simulink model "StarshipSystemModel"  (R2025b)
settings: Solver=VariableStepAuto  StartTime=0.0  StopTime=10.0  RelTol=1e-3
model workspace (MAT data in the model file):
  ActiveGNCMode : Simulink.Bus (value not decoded)
  AerodynamicControlCommand : Simulink.Bus (value not decoded)
  AerodynamicLoad : Simulink.Bus (value not decoded)
  AggregatedStream : Simulink.Bus (value not decoded)
  AllocatedEffectorDemand : Simulink.Bus (value not decoded)
  AttitudeControlDemand : Simulink.Bus (value not decoded)
  AttitudeGuidanceCommand : Simulink.Bus (value not decoded)
  AttitudeRateState : Simulink.Bus (value not decoded)
  AutogenousPressurantGas : Simulink.ConnectionBus (value not decoded)
  CandidateFaultIndication : Simulink.Bus (value not decoded)
  CombustionGasFeed : Simulink.ConnectionBus (value not decoded)
  CommandPathHealth : Simulink.Bus (value not decoded)
  ControlMode : Simulink.ValueType (value not decoded)
  DownlinkSignal : Simulink.Bus (value not decoded)
  ElectricalPower : Simulink.ConnectionBus (value not decoded)
  EngineTelemetry : Simulink.Bus (value not decoded)
  ExecutionContext : Simulink.Bus (value not decoded)
  FaultDiagnosisResult : Simulink.Bus (value not decoded)
  GNCDataContext : Simulink.Bus (value not decoded)
  GNCHealthState : Simulink.Bus (value not decoded)
  GNCStateEstimate : Simulink.Bus (value not decoded)
  GimbalAngle : Simulink.ValueType (value not decoded)
  GimbalMotion : Simulink.ConnectionBus (value not decoded)
  GroundCheckoutLink : Simulink.Bus (value not decoded)
  GroundPressurantSupply : Simulink.ConnectionBus (value not decoded)
  GuidanceConstraints : Simulink.Bus (value not decoded)
  GuidanceMode : Simulink.ValueType (value not decoded)
  LinkHealth : Simulink.Bus (value not decoded)
  LiquidPropellantFeed : Simulink.ConnectionBus (value not decoded)
  MechanicalMotion : Simulink.ConnectionBus (value not decoded)
  MechanismPosition : Simulink.Bus (value not decoded)
  ModeTransitionContext : Simulink.Bus (value not decoded)
  NavigationAidingData : Simulink.Bus (value not decoded)
  NavigationEstimate : Simulink.Bus (value not decoded)
  NavigationHealthStatus : Simulink.Bus (value not decoded)
  NavigationMeasurementSet : Simulink.Bus (value not decoded)
  PercentThrottle : Simulink.ValueType (value not decoded)
  PneumaticActuationGas : Simulink.ConnectionBus (value not decoded)
  PowerConversionStatus : Simulink.Bus (value not decoded)
  PowerDistributionStatus : Simulink.Bus (value not decoded)
  PowerHealthStatus : Simulink.Bus (value not decoded)
  PowerManagementCommand : Simulink.Bus (value not decoded)
  PowerStorageStatus : Simulink.Bus (value not decoded)
  ProtectedThermalState : Simulink.Bus (value not decoded)
  ProtectionIsolationStatus : Simulink.Bus (value not decoded)
  PurgeGasSupply : Simulink.ConnectionBus (value not decoded)
  RCSPulseCommand : Simulink.Bus (value not decoded)
  RCSTelemetry : Simulink.Bus (value not decoded)
  RFFeed : Simulink.ConnectionBus (value not decoded)
  RecoveryMechanismCommand : Simulink.Bus (value not decoded)
  RollThrottleBias : Simulink.ValueType (value not decoded)
  SafetyOverride : Simulink.ValueType (value not decoded)
  SafetyStateStatus : Simulink.Bus (value not decoded)
  ShapedControlDemand : Simulink.Bus (value not decoded)
  SpinStartIgniterGas : Simulink.ConnectionBus (value not decoded)
  StageMechanicalBoundary : Simulink.ConnectionBus (value not decoded)
  StructuralLoad : Simulink.ConnectionBus (value not decoded)
  StructureHealthStatus : Simulink.Bus (value not decoded)
  SubsystemHealthEvidence : Simulink.Bus (value not decoded)
  SubsystemStatusTelemetry : Simulink.Bus (value not decoded)
  TankTelemetry : Simulink.Bus (value not decoded)
  ThermalMonitoringCommand : Simulink.Bus (value not decoded)
  ThermalNetwork : Simulink.ConnectionBus (value not decoded)
  ThrustLoad : Simulink.ConnectionBus (value not decoded)
  TrajectoryGuidanceCommand : Simulink.Bus (value not decoded)
  TrajectoryReference : Simulink.Bus (value not decoded)
  TranslationalControlDemand : Simulink.Bus (value not decoded)
  TranslationalState : Simulink.Bus (value not decoded)
  UplinkSignal : Simulink.Bus (value not decoded)
  ValidatedControlDemand : Simulink.Bus (value not decoded)
  ValveCommand : Simulink.ValueType (value not decoded)
  VehicleStructureState : Simulink.Bus (value not decoded)
  VerifiedCommand : Simulink.Bus (value not decoded)
  VideoStream : Simulink.Bus (value not decoded)
undefined symbols (not defined in the file): ACR, ACT, ASM, ATM, BCR, BDQ, BDR, BDX, BEC, BFC, BHV, BIP, BLM, BNZ, BPI, BPR, BPV, BRX, BSM, BTA, BTP, BVC, BVE, BVV, CAA, CAM, CAS, CAT, CLM, COM, CRS, CTL, CTR, DAQ, ESC, EXT, FCR, FDB, FDE, FEX, FHI, FHM, FIC, FIS, FMG, FSC, GAP, GCM, GMD, GNC, GND, GPH, GTR, HDN, HIA, HSI, IF, INT, LOC, NAI ... (+45)
(part 6 of 8)

== system StarshipSystemModel/Starship/Thermal Protection/Thermal Barriers & Discontinuity Protection ==
  Bus Element In8 : Inport  PortName=IF-BTP-LOC-TBI-STP-01
  Bus Element In7 : Inport  Port=2  PortName=IF-BTP-FHI-TBI-INT-01
  Bus Element In6 : Inport  Port=3  PortName=IF-BTP-ACR-TBI-GAP-01
  Bus Element In5 : Inport  Port=4  PortName=IF-STP-LOC-TBI-STP-01
  Bus Element In4 : Inport  Port=5  PortName=IF-STP-CTL-TBI-CTL-01
  Bus Element In3 : Inport  Port=6  PortName=IF-STP-ACR-TBI-GAP-01
  Control-surface boundary / closeout protection : Subsystem
      settings: PortSchema="{\"entries\":[{\"content\":{\"headerSize\":26,\"margin\":15,\"minimumSpacing\":25,\"sides\":[{\"content\":{\"connectorIds\":[\"In1\"]},\"type\":\"ConnectorPlacement.EquallySpacedRectSide\",\"uuid\":\"e0cfb70a-2480-46ad-8838-78efdb61b60e\"},{\"content\":{\"connectorIds\":[\"Out1\"],\"side\":\"RIGHT\"},\"type\":\"ConnectorPlacement.EquallySpacedRectSide\",\"uuid\":\"0844e172-3ed8-42bd-94dc-a51d08e37039\"},{\"content\":{\"side\":\"TOP\"},\"type\":\"ConnectorPlacement.EquallySpacedRectSide\",\"uuid\":\"2415ea6e-ae7d-422f-a1cc-5a10cd0c87f7\"}]},\"type\":\"ConnectorPlacement.EquallySpacedConnector\",\"uuid\":\"814347a2-9201-4b2d-b96f-a93fca4a3c45\"}],\"packageUris\":[\"http://schema.mathworks.com/mf0/Connector/R2020b\"],\"version\":\"1.0\"}"
  Penetration and interface barriers : Subsystem
      settings: PortSchema="{\"entries\":[{\"content\":{\"headerSize\":26,\"margin\":15,\"minimumSpacing\":25,\"sides\":[{\"content\":{\"connectorIds\":[\"In1\"]},\"type\":\"ConnectorPlacement.EquallySpacedRectSide\",\"uuid\":\"e0cfb70a-2480-46ad-8838-78efdb61b60e\"},{\"content\":{\"connectorIds\":[\"Out1\"],\"side\":\"RIGHT\"},\"type\":\"ConnectorPlacement.EquallySpacedRectSide\",\"uuid\":\"0844e172-3ed8-42bd-94dc-a51d08e37039\"},{\"content\":{\"side\":\"TOP\"},\"type\":\"ConnectorPlacement.EquallySpacedRectSide\",\"uuid\":\"2415ea6e-ae7d-422f-a1cc-5a10cd0c87f7\"}]},\"type\":\"ConnectorPlacement.EquallySpacedConnector\",\"uuid\":\"814347a2-9201-4b2d-b96f-a93fca4a3c45\"}],\"packageUris\":[\"http://schema.mathworks.com/mf0/Connector/R2020b\"],\"version\":\"1.0\"}"
  Step / protrusion thermal management : Subsystem
      settings: PortSchema="{\"entries\":[{\"content\":{\"headerSize\":26,\"margin\":15,\"minimumSpacing\":25,\"sides\":[{\"content\":{\"connectorIds\":[\"In1\",\"In2\"]},\"type\":\"ConnectorPlacement.EquallySpacedRectSide\",\"uuid\":\"e0cfb70a-2480-46ad-8838-78efdb61b60e\"},{\"content\":{\"connectorIds\":[\"RConn1\"],\"side\":\"RIGHT\"},\"type\":\"ConnectorPlacement.EquallySpacedRectSide\",\"uuid\":\"0844e172-3ed8-42bd-94dc-a51d08e37039\"},{\"content\":{\"side\":\"TOP\"},\"type\":\"ConnectorPlacement.EquallySpacedRectSide\",\"uuid\":\"2415ea6e-ae7d-422f-a1cc-5a10cd0c87f7\"}]},\"type\":\"ConnectorPlacement.EquallySpacedConnector\",\"uuid\":\"814347a2-9201-4b2d-b96f-a93fca4a3c45\"}],\"packageUris\":[\"http://schema.mathworks.com/mf0/Connector/R2020b\"],\"version\":\"1.0\"}"
  Tile-gap / seam thermal protection : Subsystem
      settings: PortSchema="{\"entries\":[{\"content\":{\"headerSize\":26,\"margin\":15,\"minimumSpacing\":25,\"sides\":[{\"content\":{\"connectorIds\":[\"In1\",\"In2\"]},\"type\":\"ConnectorPlacement.EquallySpacedRectSide\",\"uuid\":\"e0cfb70a-2480-46ad-8838-78efdb61b60e\"},{\"content\":{\"connectorIds\":[\"Out1\"],\"side\":\"RIGHT\"},\"type\":\"ConnectorPlacement.EquallySpacedRectSide\",\"uuid\":\"0844e172-3ed8-42bd-94dc-a51d08e37039\"},{\"content\":{\"side\":\"TOP\"},\"type\":\"ConnectorPlacement.EquallySpacedRectSide\",\"uuid\":\"2415ea6e-ae7d-422f-a1cc-5a10cd0c87f7\"}]},\"type\":\"ConnectorPlacement.EquallySpacedConnector\",\"uuid\":\"814347a2-9201-4b2d-b96f-a93fca4a3c45\"}],\"packageUris\":[\"http://schema.mathworks.com/mf0/Connector/R2020b\"],\"version\":\"1.0\"}"
  IF-TBI-PRS-01 : PMIOPort  Side=Right  ConnectionType=Bus: ThermalNetwork
  Bus Element Out2 : Outport  PortName=IF-TBI-GAP-TMS-SNS-01
  Bus Element Out3 : Outport  Port=2  PortName=IF-TBI-INT-TMS-SNS-01
  Bus Element Out4 : Outport  Port=3  PortName=IF-TBI-CTL-TMS-SNS-01
  wires:
  Bus Element In4/1 -> Control-surface boundary / closeout protection/1(IF-STP-CTL-TBI-CTL-01)
  Bus Element In6/1 -> Tile-gap / seam thermal protection/1(IF-BTP-ACR-TBI-GAP-01)
  Bus Element In8/1 -> Step / protrusion thermal management/1(IF-BTP-LOC-TBI-STP-01)
  Bus Element In7/1 -> Penetration and interface barriers/1(IF-BTP-FHI-TBI-INT-01)
  Bus Element In3/1 -> Tile-gap / seam thermal protection/2(IF-STP-ACR-TBI-GAP-01)
  Bus Element In5/1 -> Step / protrusion thermal management/2(IF-STP-LOC-TBI-STP-01)
  Tile-gap / seam thermal protection/1(IF-TBI-GAP-TMS-SNS-01) -> Bus Element Out2/1
  Control-surface boundary / closeout protection/1(IF-TBI-CTL-TMS-SNS-01) -> Bus Element Out4/1
  Penetration and interface barriers/1(IF-TBI-INT-TMS-SNS-01) -> Bus Element Out3/1
  connections:
  IF-TBI-PRS-01/RConn1 -- Step / protrusion thermal management/RConn1

== system StarshipSystemModel/Starship/Thermal Protection/Thermal Monitoring & Assessment ==
  Bus Element In3 : Inport  PortName=IF-TBI-GAP-TMS-SNS-01
  Bus Element In4 : Inport  Port=2  PortName=IF-TBI-INT-TMS-SNS-01
  Bus Element In5 : Inport  Port=3  PortName=IF-TBI-CTL-TMS-SNS-01
  Bus Element In1 : Inport  Port=4  PortName=IF-GNC-TMS-01
  External thermal-observation data interface : Subsystem
      settings: PortSchema="{\"entries\":[{\"content\":{\"headerSize\":26,\"margin\":15,\"minimumSpacing\":25,\"sides\":[{\"content\":{},\"type\":\"ConnectorPlacement.EquallySpacedRectSide\",\"uuid\":\"e0cfb70a-2480-46ad-8838-78efdb61b60e\"},{\"content\":{\"connectorIds\":[\"Out1\"],\"side\":\"RIGHT\"},\"type\":\"ConnectorPlacement.EquallySpacedRectSide\",\"uuid\":\"0844e172-3ed8-42bd-94dc-a51d08e37039\"},{\"content\":{\"side\":\"TOP\"},\"type\":\"ConnectorPlacement.EquallySpacedRectSide\",\"uuid\":\"2415ea6e-ae7d-422f-a1cc-5a10cd0c87f7\"}]},\"type\":\"ConnectorPlacement.EquallySpacedConnector\",\"uuid\":\"814347a2-9201-4b2d-b96f-a93fca4a3c45\"}],\"packageUris\":[\"http://schema.mathworks.com/mf0/Connector/R2020b\"],\"version\":\"1.0\"}"
  TPS thermal sensors : Subsystem
      settings: PortSchema="{\"entries\":[{\"content\":{\"headerSize\":26,\"margin\":15,\"minimumSpacing\":25,\"sides\":[{\"content\":{\"connectorIds\":[\"In1\",\"In2\",\"In3\",\"In4\",\"LConn1\"]},\"type\":\"ConnectorPlacement.EquallySpacedRectSide\",\"uuid\":\"e0cfb70a-2480-46ad-8838-78efdb61b60e\"},{\"content\":{\"connectorIds\":[\"Out1\"],\"side\":\"RIGHT\"},\"type\":\"ConnectorPlacement.EquallySpacedRectSide\",\"uuid\":\"0844e172-3ed8-42bd-94dc-a51d08e37039\"},{\"content\":{\"side\":\"TOP\"},\"type\":\"ConnectorPlacement.EquallySpacedRectSide\",\"uuid\":\"2415ea6e-ae7d-422f-a1cc-5a10cd0c87f7\"}]},\"type\":\"ConnectorPlacement.EquallySpacedConnector\",\"uuid\":\"814347a2-9201-4b2d-b96f-a93fca4a3c45\"}],\"packageUris\":[\"http://schema.mathworks.com/mf0/Connector/R2020b\"],\"version\":\"1.0\"}"
  Thermal assessment / reconstruction function : Subsystem
      settings: PortSchema="{\"entries\":[{\"content\":{\"headerSize\":26,\"margin\":15,\"minimumSpacing\":25,\"sides\":[{\"content\":{\"connectorIds\":[\"In1\",\"In2\"]},\"type\":\"ConnectorPlacement.EquallySpacedRectSide\",\"uuid\":\"e0cfb70a-2480-46ad-8838-78efdb61b60e\"},{\"content\":{\"connectorIds\":[\"Out1\"],\"side\":\"RIGHT\"},\"type\":\"ConnectorPlacement.EquallySpacedRectSide\",\"uuid\":\"0844e172-3ed8-42bd-94dc-a51d08e37039\"},{\"content\":{\"side\":\"TOP\"},\"type\":\"ConnectorPlacement.EquallySpacedRectSide\",\"uuid\":\"2415ea6e-ae7d-422f-a1cc-5a10cd0c87f7\"}]},\"type\":\"ConnectorPlacement.EquallySpacedConnector\",\"uuid\":\"814347a2-9201-4b2d-b96f-a93fca4a3c45\"}],\"packageUris\":[\"http://schema.mathworks.com/mf0/Connector/R2020b\"],\"version\":\"1.0\"}"
  Thermal-data acquisition / telemetry path : Subsystem
      settings: PortSchema="{\"entries\":[{\"content\":{\"headerSize\":26,\"margin\":15,\"minimumSpacing\":25,\"sides\":[{\"content\":{\"connectorIds\":[\"In1\",\"In2\"]},\"type\":\"ConnectorPlacement.EquallySpacedRectSide\",\"uuid\":\"e0cfb70a-2480-46ad-8838-78efdb61b60e\"},{\"content\":{\"connectorIds\":[\"Out1\"],\"side\":\"RIGHT\"},\"type\":\"ConnectorPlacement.EquallySpacedRectSide\",\"uuid\":\"0844e172-3ed8-42bd-94dc-a51d08e37039\"},{\"content\":{\"side\":\"TOP\"},\"type\":\"ConnectorPlacement.EquallySpacedRectSide\",\"uuid\":\"2415ea6e-ae7d-422f-a1cc-5a10cd0c87f7\"}]},\"type\":\"ConnectorPlacement.EquallySpacedConnector\",\"uuid\":\"814347a2-9201-4b2d-b96f-a93fca4a3c45\"}],\"packageUris\":[\"http://schema.mathworks.com/mf0/Connector/R2020b\"],\"version\":\"1.0\"}"
  IF-PWR-TMS-01 : PMIOPort  Side=Left  ConnectionType=Bus: ElectricalPower
  Bus Element Out1 : Outport  PortName=IF-TMS-GNC-01
  Bus Element Out2 : Outport  Port=2  PortName=IF-TMS-BTA-01
  Bus Element Out3 : Outport  Port=3  PortName=IF-TMS-STA-01
  Bus Element Out4 : Outport  Port=4  PortName=IF-TMS-SAF-01
  wires:
  Bus Element In3/1 -> TPS thermal sensors/1(IF-TBI-GAP-TMS-SNS-01)
  Bus Element In4/1 -> TPS thermal sensors/2(IF-TBI-INT-TMS-SNS-01)
  Bus Element In5/1 -> TPS thermal sensors/3(IF-TBI-CTL-TMS-SNS-01)
  TPS thermal sensors/1(IF-TMS-SNS-DAQ-01) -> Thermal-data acquisition / telemetry path/1(IF-TMS-SNS-DAQ-01)
  Thermal-data acquisition / telemetry path/1(IF-TMS-DAQ-ASM-01) -> Thermal assessment / reconstruction function/1(IF-TMS-DAQ-ASM-01)
  Thermal assessment / reconstruction function/1(IF-TMS-ASM-DAQ-01) -> Thermal-data acquisition / telemetry path/2(IF-TMS-ASM-DAQ-01)
  External thermal-observation data interface/1(IF-TMS-EXT-ASM-01) -> Thermal assessment / reconstruction function/2(IF-TMS-EXT-ASM-01)
  Bus Element In1/1 -> TPS thermal sensors/4(IF-GNC-TMS-01)
  connections:
  IF-PWR-TMS-01/RConn1 -- TPS thermal sensors/LConn1

== system StarshipSystemModel/Starship/Communications/Booster/Command & Data Handling (C&DH) ==
  Bus Element In6 : Inport  PortName=IF-INT-BTA-01
  Bus Element In5 : Inport  Port=2  PortName=IF-TMS-BTA-01
  Bus Element In9 : Inport  Port=3  PortName=IF-BDQ-BCR-01
  Bus Element In8 : Inport  Port=4  PortName=IF-BDX-BLM-01
  Bus Element In7 : Inport  Port=5  PortName=IF-BRX-BLM-01
  Bus Element In3 : Inport  Port=6  PortName=IF-GNC-BTA-01
  Bus Element In2 : Inport  Port=7  PortName=IF-BPR-BTA-01
  Bus Element In1 : Inport  Port=8  PortName=IF-BEC-BTA-01
  Bus Element In4 : Inport  Port=9  PortName=IF-SAF-BTA-01
  Command decoder & router : Subsystem
      settings: PortSchema="{\"entries\":[{\"content\":{\"headerSize\":26,\"margin\":15,\"minimumSpacing\":25,\"sides\":[{\"content\":{\"connectorIds\":[\"In1\",\"In2\"]},\"type\":\"ConnectorPlacement.EquallySpacedRectSide\",\"uuid\":\"57d8a002-ec9a-4125-b797-7e7c6712bf02\"},{\"content\":{\"connectorIds\":[\"Out1\",\"Out2\"],\"side\":\"RIGHT\"},\"type\":\"ConnectorPlacement.EquallySpacedRectSide\",\"uuid\":\"9c166a96-12fc-4382-8ebe-da88da7fda26\"},{\"content\":{\"side\":\"TOP\"},\"type\":\"ConnectorPlacement.EquallySpacedRectSide\",\"uuid\":\"d709cb41-f5aa-4a2a-ad2b-35894222a9c1\"}]},\"type\":\"ConnectorPlacement.EquallySpacedConnector\",\"uuid\":\"04bb3772-118b-42d1-ac15-43c1b901053a\"}],\"packageUris\":[\"http://schema.mathworks.com/mf0/Connector/R2020b\"],\"version\":\"1.0\"}"
  Data recorder (mass memory) : Subsystem
      settings: PortSchema="{\"entries\":[{\"content\":{\"headerSize\":26,\"margin\":15,\"minimumSpacing\":25,\"sides\":[{\"content\":{\"connectorIds\":[\"In1\"]},\"type\":\"ConnectorPlacement.EquallySpacedRectSide\",\"uuid\":\"57d8a002-ec9a-4125-b797-7e7c6712bf02\"},{\"content\":{\"side\":\"RIGHT\"},\"type\":\"ConnectorPlacement.EquallySpacedRectSide\",\"uuid\":\"9c166a96-12fc-4382-8ebe-da88da7fda26\"},{\"content\":{\"side\":\"TOP\"},\"type\":\"ConnectorPlacement.EquallySpacedRectSide\",\"uuid\":\"d709cb41-f5aa-4a2a-ad2b-35894222a9c1\"}]},\"type\":\"ConnectorPlacement.EquallySpacedConnector\",\"uuid\":\"04bb3772-118b-42d1-ac15-43c1b901053a\"}],\"packageUris\":[\"http://schema.mathworks.com/mf0/Connector/R2020b\"],\"version\":\"1.0\"}"
  Link management controller : Subsystem
      settings: PortSchema="{\"entries\":[{\"content\":{\"headerSize\":26,\"margin\":15,\"minimumSpacing\":25,\"sides\":[{\"content\":{\"connectorIds\":[\"In1\",\"In2\",\"In3\"]},\"type\":\"ConnectorPlacement.EquallySpacedRectSide\",\"uuid\":\"57d8a002-ec9a-4125-b797-7e7c6712bf02\"},{\"content\":{\"connectorIds\":[\"Out1\",\"Out2\",\"Out3\",\"Out4\"],\"side\":\"RIGHT\"},\"type\":\"ConnectorPlacement.EquallySpacedRectSide\",\"uuid\":\"9c166a96-12fc-4382-8ebe-da88da7fda26\"},{\"content\":{\"side\":\"TOP\"},\"type\":\"ConnectorPlacement.EquallySpacedRectSide\",\"uuid\":\"d709cb41-f5aa-4a2a-ad2b-35894222a9c1\"}]},\"type\":\"ConnectorPlacement.EquallySpacedConnector\",\"uuid\":\"04bb3772-118b-42d1-ac15-43c1b901053a\"}],\"packageUris\":[\"http://schema.mathworks.com/mf0/Connector/R2020b\"],\"version\":\"1.0\"}"
  Telemetry aggregator : Subsystem
      settings: PortSchema="{\"entries\":[{\"content\":{\"headerSize\":26,\"margin\":15,\"minimumSpacing\":25,\"sides\":[{\"content\":{\"connectorIds\":[\"LConn1\",\"In1\",\"In2\",\"In3\",\"In4\",\"In5\",\"In7\",\"In6\"]},\"type\":\"ConnectorPlacement.EquallySpacedRectSide\",\"uuid\":\"57d8a002-ec9a-4125-b797-7e7c6712bf02\"},{\"content\":{\"connectorIds\":[\"Out1\",\"Out2\",\"Out3\"],\"side\":\"RIGHT\"},\"type\":\"ConnectorPlacement.EquallySpacedRectSide\",\"uuid\":\"9c166a96-12fc-4382-8ebe-da88da7fda26\"},{\"content\":{\"side\":\"TOP\"},\"type\":\"ConnectorPlacement.EquallySpacedRectSide\",\"uuid\":\"d709cb41-f5aa-4a2a-ad2b-35894222a9c1\"}]},\"type\":\"ConnectorPlacement.EquallySpacedConnector\",\"uuid\":\"04bb3772-118b-42d1-ac15-43c1b901053a\"}],\"packageUris\":[\"http://schema.mathworks.com/mf0/Connector/R2020b\"],\"version\":\"1.0\"}"
  Video capture & encoding : Subsystem
      settings: PortSchema="{\"entries\":[{\"content\":{\"headerSize\":26,\"margin\":15,\"minimumSpacing\":25,\"sides\":[{\"content\":{},\"type\":\"ConnectorPlacement.EquallySpacedRectSide\",\"uuid\":\"57d8a002-ec9a-4125-b797-7e7c6712bf02\"},{\"content\":{\"connectorIds\":[\"Out1\"],\"side\":\"RIGHT\"},\"type\":\"ConnectorPlacement.EquallySpacedRectSide\",\"uuid\":\"9c166a96-12fc-4382-8ebe-da88da7fda26\"},{\"content\":{\"side\":\"TOP\"},\"type\":\"ConnectorPlacement.EquallySpacedRectSide\",\"uuid\":\"d709cb41-f5aa-4a2a-ad2b-35894222a9c1\"}]},\"type\":\"ConnectorPlacement.EquallySpacedConnector\",\"uuid\":\"04bb3772-118b-42d1-ac15-43c1b901053a\"}],\"packageUris\":[\"http://schema.mathworks.com/mf0/Connector/R2020b\"],\"version\":\"1.0\"}"
  IF-PWR-BTA-01 : PMIOPort  Side=Left  ConnectionType=Bus: ElectricalPower
  Bus Element Out6 : Outport  PortName=IF-BTA-BDQ-01
  Bus Element Out1 : Outport  Port=2  PortName=IF-BCR-GNC-01
  Bus Element Out3 : Outport  Port=3  PortName=IF-BLM-SAF-01
  Bus Element Out2 : Outport  Port=4  PortName=IF-BCR-SAF-01
  Bus Element Out4 : Outport  Port=5  PortName=IF-BLM-BRX-01
  Bus Element Out5 : Outport  Port=6  PortName=IF-BLM-BDX-01
  wires:
  Bus Element In8/1 -> Link management controller/3(IF-BDX-BLM-01)
  Bus Element In3/1 -> Telemetry aggregator/3(IF-GNC-BTA-01)
  Bus Element In9/1 -> Command decoder & router/1(IF-BDQ-BCR-01)
  Bus Element In7/1 -> Link management controller/2(IF-BRX-BLM-01)
  Command decoder & router/1(IF-BCR-GNC-01) -> Bus Element Out1/1
  Bus Element In2/1 -> Telemetry aggregator/5(IF-BPR-BTA-01)
  Bus Element In4/1 -> Telemetry aggregator/7(IF-SAF-BTA-01)
  Bus Element In1/1 -> Telemetry aggregator/4(IF-BEC-BTA-01)
  Video capture & encoding/1(IF-BVE-BTA-01) -> Telemetry aggregator/6(IF-BVE-BTA-01)
  Telemetry aggregator/1(IF-BTA-BLM-01) -> Link management controller/1(IF-BTA-BLM-01)
  Telemetry aggregator/2(IF-BTA-BDR-01) -> Data recorder (mass memory)/1(IF-BTA-BDR-01)
  Telemetry aggregator/3(IF-BTA-BDQ-01) -> Bus Element Out6/1
  Link management controller/1(IF-BLM-SAF-01) -> Bus Element Out3/1
  Link management controller/2(IF-BLM-BRX-01) -> Bus Element Out4/1
  Link management controller/3(IF-BLM-BDX-01) -> Bus Element Out5/1
  Link management controller/4(IF-BLM-BCR-01) -> Command decoder & router/2(IF-BLM-BCR-01)
  Command decoder & router/2(IF-BCR-SAF-01) -> Bus Element Out2/1
  Bus Element In5/1 -> Telemetry aggregator/2(IF-TMS-BTA-01)
  Bus Element In6/1 -> Telemetry aggregator/1(IF-INT-BTA-01)
  connections:
  IF-PWR-BTA-01/RConn1 -- Telemetry aggregator/LConn1

== system StarshipSystemModel/Starship/Communications/Booster/Direct-to-ground RF terminal ==
  Bus Element In1 : Inport  PortName=IF-GND-BDX-01
  Bus Element In2 : Inport  Port=2  PortName=IF-BLM-BDX-01
  Antenna array : Subsystem
      settings: PortSchema="{\"entries\":[{\"content\":{\"headerSize\":26,\"margin\":15,\"minimumSpacing\":25,\"sides\":[{\"content\":{},\"type\":\"ConnectorPlacement.EquallySpacedRectSide\",\"uuid\":\"57d8a002-ec9a-4125-b797-7e7c6712bf02\"},{\"content\":{\"connectorIds\":[\"RConn1\"],\"side\":\"RIGHT\"},\"type\":\"ConnectorPlacement.EquallySpacedRectSide\",\"uuid\":\"9c166a96-12fc-4382-8ebe-da88da7fda26\"},{\"content\":{\"side\":\"TOP\"},\"type\":\"ConnectorPlacement.EquallySpacedRectSide\",\"uuid\":\"d709cb41-f5aa-4a2a-ad2b-35894222a9c1\"}]},\"type\":\"ConnectorPlacement.EquallySpacedConnector\",\"uuid\":\"04bb3772-118b-42d1-ac15-43c1b901053a\"}],\"packageUris\":[\"http://schema.mathworks.com/mf0/Connector/R2020b\"],\"version\":\"1.0\"}"
  RF transceiver unit : Subsystem
      settings: PortSchema="{\"entries\":[{\"content\":{\"headerSize\":26,\"margin\":15,\"minimumSpacing\":25,\"sides\":[{\"content\":{\"connectorIds\":[\"LConn1\",\"In1\",\"LConn2\",\"In2\"]},\"type\":\"ConnectorPlacement.EquallySpacedRectSide\",\"uuid\":\"57d8a002-ec9a-4125-b797-7e7c6712bf02\"},{\"content\":{\"connectorIds\":[\"Out1\",\"Out2\"],\"side\":\"RIGHT\"},\"type\":\"ConnectorPlacement.EquallySpacedRectSide\",\"uuid\":\"9c166a96-12fc-4382-8ebe-da88da7fda26\"},{\"content\":{\"side\":\"TOP\"},\"type\":\"ConnectorPlacement.EquallySpacedRectSide\",\"uuid\":\"d709cb41-f5aa-4a2a-ad2b-35894222a9c1\"}]},\"type\":\"ConnectorPlacement.EquallySpacedConnector\",\"uuid\":\"04bb3772-118b-42d1-ac15-43c1b901053a\"}],\"packageUris\":[\"http://schema.mathworks.com/mf0/Connector/R2020b\"],\"version\":\"1.0\"}"
  IF-PWR-BDX-01 : PMIOPort  Side=Left  ConnectionType=Bus: ElectricalPower
  Bus Element Out1 : Outport  PortName=IF-BDX-GND-01
  Bus Element Out2 : Outport  Port=2  PortName=IF-BDX-BLM-01
  wires:
  Bus Element In1/1 -> RF transceiver unit/1(IF-GND-BDX-01)
  RF transceiver unit/1(IF-BDX-GND-01) -> Bus Element Out1/1
  Bus Element In2/1 -> RF transceiver unit/2(IF-BLM-BDX-01)
  RF transceiver unit/2(IF-BDX-BLM-01) -> Bus Element Out2/1
  connections:
  Antenna array/RConn1 -- RF transceiver unit/LConn2
  IF-PWR-BDX-01/RConn1 -- RF transceiver unit/LConn1

== system StarshipSystemModel/Starship/Communications/Booster/Ground data interface ==
  Bus Element In2 : Inport  PortName=IF-BTA-BDQ-01
  Bus Element In1 : Inport  Port=2  PortName=IF-GND-BDQ-01
  Vehicle-side data QD panel : Subsystem
      settings: PortSchema="{\"entries\":[{\"content\":{\"headerSize\":26,\"margin\":15,\"minimumSpacing\":25,\"sides\":[{\"content\":{\"connectorIds\":[\"In1\",\"In2\"]},\"type\":\"ConnectorPlacement.EquallySpacedRectSide\",\"uuid\":\"57d8a002-ec9a-4125-b797-7e7c6712bf02\"},{\"content\":{\"connectorIds\":[\"Out1\",\"Out2\"],\"side\":\"RIGHT\"},\"type\":\"ConnectorPlacement.EquallySpacedRectSide\",\"uuid\":\"9c166a96-12fc-4382-8ebe-da88da7fda26\"},{\"content\":{\"side\":\"TOP\"},\"type\":\"ConnectorPlacement.EquallySpacedRectSide\",\"uuid\":\"d709cb41-f5aa-4a2a-ad2b-35894222a9c1\"}]},\"type\":\"ConnectorPlacement.EquallySpacedConnector\",\"uuid\":\"04bb3772-118b-42d1-ac15-43c1b901053a\"}],\"packageUris\":[\"http://schema.mathworks.com/mf0/Connector/R2020b\"],\"version\":\"1.0\"}"
  Bus Element Out1 : Outport  PortName=IF-BDQ-GND-01
  Bus Element Out2 : Outport  Port=2  PortName=IF-BDQ-BCR-01
  wires:
  Bus Element In1/1 -> Vehicle-side data QD panel/2(IF-GND-BDQ-01)
  Vehicle-side data QD panel/1("IF-BDQ-GND-01\t") -> Bus Element Out1/1
  Vehicle-side data QD panel/2(IF-BDQ-BCR-01) -> Bus Element Out2/1
  Bus Element In2/1 -> Vehicle-side data QD panel/1(IF-BTA-BDQ-01)

== system StarshipSystemModel/Starship/Communications/Booster/Relay link terminal ==
  Bus Element In1 : Inport  PortName=IF-GND-BRX-01
  Bus Element In2 : Inport  Port=2  PortName=IF-BLM-BRX-01
  Antenna aperture & radome : Subsystem
      settings: PortSchema="{\"entries\":[{\"content\":{\"headerSize\":26,\"margin\":15,\"minimumSpacing\":25,\"sides\":[{\"content\":{\"connectorIds\":[\"LConn1\"]},\"type\":\"ConnectorPlacement.EquallySpacedRectSide\",\"uuid\":\"57d8a002-ec9a-4125-b797-7e7c6712bf02\"},{\"content\":{\"connectorIds\":[\"RConn1\"],\"side\":\"RIGHT\"},\"type\":\"ConnectorPlacement.EquallySpacedRectSide\",\"uuid\":\"9c166a96-12fc-4382-8ebe-da88da7fda26\"},{\"content\":{\"side\":\"TOP\"},\"type\":\"ConnectorPlacement.EquallySpacedRectSide\",\"uuid\":\"d709cb41-f5aa-4a2a-ad2b-35894222a9c1\"}]},\"type\":\"ConnectorPlacement.EquallySpacedConnector\",\"uuid\":\"04bb3772-118b-42d1-ac15-43c1b901053a\"}],\"packageUris\":[\"http://schema.mathworks.com/mf0/Connector/R2020b\"],\"version\":\"1.0\"}"
  RF/optical transceiver unit : Subsystem
      settings: PortSchema="{\"entries\":[{\"content\":{\"headerSize\":26,\"margin\":15,\"minimumSpacing\":25,\"sides\":[{\"content\":{\"connectorIds\":[\"In1\",\"LConn1\",\"In2\",\"LConn2\"]},\"type\":\"ConnectorPlacement.EquallySpacedRectSide\",\"uuid\":\"57d8a002-ec9a-4125-b797-7e7c6712bf02\"},{\"content\":{\"connectorIds\":[\"Out1\",\"Out2\"],\"side\":\"RIGHT\"},\"type\":\"ConnectorPlacement.EquallySpacedRectSide\",\"uuid\":\"9c166a96-12fc-4382-8ebe-da88da7fda26\"},{\"content\":{\"side\":\"TOP\"},\"type\":\"ConnectorPlacement.EquallySpacedRectSide\",\"uuid\":\"d709cb41-f5aa-4a2a-ad2b-35894222a9c1\"}]},\"type\":\"ConnectorPlacement.EquallySpacedConnector\",\"uuid\":\"04bb3772-118b-42d1-ac15-43c1b901053a\"}],\"packageUris\":[\"http://schema.mathworks.com/mf0/Connector/R2020b\"],\"version\":\"1.0\"}"
  IF-PWR-BRA-01 : PMIOPort  Side=Left  ConnectionType=Bus: ElectricalPower
  IF-PWR-BRX-01 : PMIOPort  Port=2  Side=Left  ConnectionType=Bus: ElectricalPower
  Bus Element Out1 : Outport  PortName=IF-BRX-GND-01
  Bus Element Out2 : Outport  Port=2  PortName=IF-BRX-BLM-01
  wires:
  Bus Element In1/1 -> RF/optical transceiver unit/1(IF-GND-BRX-01)
  RF/optical transceiver unit/1(IF-BRX-GND-01) -> Bus Element Out1/1
  Bus Element In2/1 -> RF/optical transceiver unit/2(IF-BLM-BRX-01)
  RF/optical transceiver unit/2(IF-BRX-BLM-01) -> Bus Element Out2/1
  connections:
  Antenna aperture & radome/RConn1 -- RF/optical transceiver unit/LConn1
  IF-PWR-BRA-01/RConn1 -- Antenna aperture & radome/LConn1
  IF-PWR-BRX-01/RConn1 -- RF/optical transceiver unit/LConn2

== system StarshipSystemModel/Starship/Communications/Ship/Command & Data Handling (C&DH) ==
  Bus Element In5 : Inport  PortName=IF-TMS-STA-01
  Bus Element In9 : Inport  Port=2  PortName=IF-SDQ-SCR-01
  Bus Element In8 : Inport  Port=3  PortName=IF-SDX-SLM-01
  Bus Element In7 : Inport  Port=4  PortName=IF-SRX-SLM-01
  Bus Element In3 : Inport  Port=5  PortName=IF-GNC-STA-01
  Bus Element In2 : Inport  Port=6  PortName=IF-SPR-STA-01
  Bus Element In1 : Inport  Port=7  PortName=IF-SEC-STA-01
  Bus Element In4 : Inport  Port=8  PortName=IF-SAF-STA-01
  Bus Element In6 : Inport  Port=9  PortName=IF-INT-STA-01
  Command decoder & router : Subsystem
      settings: PortSchema="{\"entries\":[{\"content\":{\"headerSize\":26,\"margin\":15,\"minimumSpacing\":25,\"sides\":[{\"content\":{\"connectorIds\":[\"In1\",\"In2\"]},\"type\":\"ConnectorPlacement.EquallySpacedRectSide\",\"uuid\":\"57d8a002-ec9a-4125-b797-7e7c6712bf02\"},{\"content\":{\"connectorIds\":[\"Out1\",\"Out2\"],\"side\":\"RIGHT\"},\"type\":\"ConnectorPlacement.EquallySpacedRectSide\",\"uuid\":\"9c166a96-12fc-4382-8ebe-da88da7fda26\"},{\"content\":{\"side\":\"TOP\"},\"type\":\"ConnectorPlacement.EquallySpacedRectSide\",\"uuid\":\"d709cb41-f5aa-4a2a-ad2b-35894222a9c1\"}]},\"type\":\"ConnectorPlacement.EquallySpacedConnector\",\"uuid\":\"04bb3772-118b-42d1-ac15-43c1b901053a\"}],\"packageUris\":[\"http://schema.mathworks.com/mf0/Connector/R2020b\"],\"version\":\"1.0\"}"
  Data recorder (mass memory) : Subsystem
      settings: PortSchema="{\"entries\":[{\"content\":{\"headerSize\":26,\"margin\":15,\"minimumSpacing\":25,\"sides\":[{\"content\":{\"connectorIds\":[\"In1\"]},\"type\":\"ConnectorPlacement.EquallySpacedRectSide\",\"uuid\":\"57d8a002-ec9a-4125-b797-7e7c6712bf02\"},{\"content\":{\"side\":\"RIGHT\"},\"type\":\"ConnectorPlacement.EquallySpacedRectSide\",\"uuid\":\"9c166a96-12fc-4382-8ebe-da88da7fda26\"},{\"content\":{\"side\":\"TOP\"},\"type\":\"ConnectorPlacement.EquallySpacedRectSide\",\"uuid\":\"d709cb41-f5aa-4a2a-ad2b-35894222a9c1\"}]},\"type\":\"ConnectorPlacement.EquallySpacedConnector\",\"uuid\":\"04bb3772-118b-42d1-ac15-43c1b901053a\"}],\"packageUris\":[\"http://schema.mathworks.com/mf0/Connector/R2020b\"],\"version\":\"1.0\"}"
  Link management controller : Subsystem
      settings: PortSchema="{\"entries\":[{\"content\":{\"headerSize\":26,\"margin\":15,\"minimumSpacing\":25,\"sides\":[{\"content\":{\"connectorIds\":[\"In1\",\"In2\",\"In3\"]},\"type\":\"ConnectorPlacement.EquallySpacedRectSide\",\"uuid\":\"57d8a002-ec9a-4125-b797-7e7c6712bf02\"},{\"content\":{\"connectorIds\":[\"Out1\",\"Out2\",\"Out3\",\"Out4\"],\"side\":\"RIGHT\"},\"type\":\"ConnectorPlacement.EquallySpacedRectSide\",\"uuid\":\"9c166a96-12fc-4382-8ebe-da88da7fda26\"},{\"content\":{\"side\":\"TOP\"},\"type\":\"ConnectorPlacement.EquallySpacedRectSide\",\"uuid\":\"d709cb41-f5aa-4a2a-ad2b-35894222a9c1\"}]},\"type\":\"ConnectorPlacement.EquallySpacedConnector\",\"uuid\":\"04bb3772-118b-42d1-ac15-43c1b901053a\"}],\"packageUris\":[\"http://schema.mathworks.com/mf0/Connector/R2020b\"],\"version\":\"1.0\"}"
  Telemetry aggregator : Subsystem
      settings: PortSchema="{\"entries\":[{\"content\":{\"headerSize\":26,\"margin\":15,\"minimumSpacing\":25,\"sides\":[{\"content\":{\"connectorIds\":[\"LConn1\",\"In1\",\"In2\",\"In3\",\"In4\",\"In6\",\"In5\",\"In7\"]},\"type\":\"ConnectorPlacement.EquallySpacedRectSide\",\"uuid\":\"57d8a002-ec9a-4125-b797-7e7c6712bf02\"},{\"content\":{\"connectorIds\":[\"Out1\",\"Out2\",\"Out3\"],\"side\":\"RIGHT\"},\"type\":\"ConnectorPlacement.EquallySpacedRectSide\",\"uuid\":\"9c166a96-12fc-4382-8ebe-da88da7fda26\"},{\"content\":{\"side\":\"TOP\"},\"type\":\"ConnectorPlacement.EquallySpacedRectSide\",\"uuid\":\"d709cb41-f5aa-4a2a-ad2b-35894222a9c1\"}]},\"type\":\"ConnectorPlacement.EquallySpacedConnector\",\"uuid\":\"04bb3772-118b-42d1-ac15-43c1b901053a\"}],\"packageUris\":[\"http://schema.mathworks.com/mf0/Connector/R2020b\"],\"version\":\"1.0\"}"
  Video capture & encoding : Subsystem
      settings: PortSchema="{\"entries\":[{\"content\":{\"headerSize\":26,\"margin\":15,\"minimumSpacing\":25,\"sides\":[{\"content\":{},\"type\":\"ConnectorPlacement.EquallySpacedRectSide\",\"uuid\":\"57d8a002-ec9a-4125-b797-7e7c6712bf02\"},{\"content\":{\"connectorIds\":[\"Out1\"],\"side\":\"RIGHT\"},\"type\":\"ConnectorPlacement.EquallySpacedRectSide\",\"uuid\":\"9c166a96-12fc-4382-8ebe-da88da7fda26\"},{\"content\":{\"side\":\"TOP\"},\"type\":\"ConnectorPlacement.EquallySpacedRectSide\",\"uuid\":\"d709cb41-f5aa-4a2a-ad2b-35894222a9c1\"}]},\"type\":\"ConnectorPlacement.EquallySpacedConnector\",\"uuid\":\"04bb3772-118b-42d1-ac15-43c1b901053a\"}],\"packageUris\":[\"http://schema.mathworks.com/mf0/Connector/R2020b\"],\"version\":\"1.0\"}"
  IF-PWR-STA-01 : PMIOPort  Side=Left  ConnectionType=Bus: ElectricalPower
  Bus Element Out6 : Outport  PortName=IF-STA-SDQ-01
  Bus Element Out2 : Outport  Port=2  PortName=IF-SCR-SAF-01
  Bus Element Out3 : Outport  Port=3  PortName=IF-SLM-SAF-01
  Bus Element Out1 : Outport  Port=4  PortName=IF-SCR-GNC-01
  Bus Element Out4 : Outport  Port=5  PortName=IF-SLM-SRX-01
  Bus Element Out5 : Outport  Port=6  PortName=IF-SLM-SDX-01
  wires:
  Telemetry aggregator/2(IF-STA-SDR-01) -> Data recorder (mass memory)/1(IF-STA-SDR-01)
  Bus Element In4/1 -> Telemetry aggregator/6(IF-SAF-STA-01)
  Bus Element In2/1 -> Telemetry aggregator/4(IF-SPR-STA-01)
  Bus Element In1/1 -> Telemetry aggregator/3(IF-SEC-STA-01)
  Bus Element In3/1 -> Telemetry aggregator/2(IF-GNC-STA-01)
  Video capture & encoding/1(IF-SVE-STA-01) -> Telemetry aggregator/5(IF-SVE-STA-01)
  Command decoder & router/2(IF-SCR-SAF-01) -> Bus Element Out2/1
  Telemetry aggregator/1(IF-STA-SLM-01) -> Link management controller/1(IF-STA-SLM-01)
  Telemetry aggregator/3(IF-STA-SDQ-01) -> Bus Element Out6/1
  Bus Element In7/1 -> Link management controller/2(IF-SRX-SLM-01)
  Bus Element In8/1 -> Link management controller/3(IF-SDX-SLM-01)
  Link management controller/1(IF-SLM-SAF-01) -> Bus Element Out3/1
  Link management controller/2(IF-SLM-SRX-01) -> Bus Element Out4/1
  Link management controller/3(IF-SLM-SDX-01) -> Bus Element Out5/1
  Link management controller/4(IF-SLM-SCR-01) -> Command decoder & router/2(IF-SLM-SCR-01)
  Bus Element In9/1 -> Command decoder & router/1(IF-SDQ-SCR-01)
  Command decoder & router/1(IF-SCR-GNC-01) -> Bus Element Out1/1
  Bus Element In5/1 -> Telemetry aggregator/1(IF-TMS-STA-01)
  Bus Element In6/1 -> Telemetry aggregator/7(IF-INT-STA-01)
  connections:
  IF-PWR-STA-01/RConn1 -- Telemetry aggregator/LConn1

== system StarshipSystemModel/Starship/Communications/Ship/Direct-to-ground RF terminal ==
  Bus Element In1 : Inport  PortName=IF-GND-SDX-01
  Bus Element In2 : Inport  Port=2  PortName=IF-SLM-SDX-01
  Antenna array : Subsystem
      settings: PortSchema="{\"entries\":[{\"content\":{\"headerSize\":26,\"margin\":15,\"minimumSpacing\":25,\"sides\":[{\"content\":{},\"type\":\"ConnectorPlacement.EquallySpacedRectSide\",\"uuid\":\"57d8a002-ec9a-4125-b797-7e7c6712bf02\"},{\"content\":{\"connectorIds\":[\"RConn1\"],\"side\":\"RIGHT\"},\"type\":\"ConnectorPlacement.EquallySpacedRectSide\",\"uuid\":\"9c166a96-12fc-4382-8ebe-da88da7fda26\"},{\"content\":{\"side\":\"TOP\"},\"type\":\"ConnectorPlacement.EquallySpacedRectSide\",\"uuid\":\"d709cb41-f5aa-4a2a-ad2b-35894222a9c1\"}]},\"type\":\"ConnectorPlacement.EquallySpacedConnector\",\"uuid\":\"04bb3772-118b-42d1-ac15-43c1b901053a\"}],\"packageUris\":[\"http://schema.mathworks.com/mf0/Connector/R2020b\"],\"version\":\"1.0\"}"
  RF transceiver unit : Subsystem
      settings: PortSchema="{\"entries\":[{\"content\":{\"headerSize\":26,\"margin\":15,\"minimumSpacing\":25,\"sides\":[{\"content\":{\"connectorIds\":[\"LConn1\",\"In1\",\"LConn2\",\"In2\"]},\"type\":\"ConnectorPlacement.EquallySpacedRectSide\",\"uuid\":\"57d8a002-ec9a-4125-b797-7e7c6712bf02\"},{\"content\":{\"connectorIds\":[\"Out1\",\"Out2\"],\"side\":\"RIGHT\"},\"type\":\"ConnectorPlacement.EquallySpacedRectSide\",\"uuid\":\"9c166a96-12fc-4382-8ebe-da88da7fda26\"},{\"content\":{\"side\":\"TOP\"},\"type\":\"ConnectorPlacement.EquallySpacedRectSide\",\"uuid\":\"d709cb41-f5aa-4a2a-ad2b-35894222a9c1\"}]},\"type\":\"ConnectorPlacement.EquallySpacedConnector\",\"uuid\":\"04bb3772-118b-42d1-ac15-43c1b901053a\"}],\"packageUris\":[\"http://schema.mathworks.com/mf0/Connector/R2020b\"],\"version\":\"1.0\"}"
  IF-PWR-SDX-01 : PMIOPort  Side=Left  ConnectionType=Bus: ElectricalPower
  Bus Element Out1 : Outport  PortName=IF-SDX-GND-01
  Bus Element Out2 : Outport  Port=2  PortName=IF-SDX-SLM-01
  wires:
  RF transceiver unit/1(IF-SDX-GND-01) -> Bus Element Out1/1
  Bus Element In1/1 -> RF transceiver unit/1(IF-GND-SDX-01)
  Bus Element In2/1 -> RF transceiver unit/2(IF-SLM-SDX-01)
  RF transceiver unit/2(IF-SDX-SLM-01) -> Bus Element Out2/1
  connections:
  Antenna array/RConn1 -- RF transceiver unit/LConn2
  IF-PWR-SDX-01/RConn1 -- RF transceiver unit/LConn1

== system StarshipSystemModel/Starship/Communications/Ship/Ground data interface ==
  Bus Element In2 : Inport  PortName=IF-STA-SDQ-01
  Bus Element In1 : Inport  Port=2  PortName=IF-GND-SDQ-01
  Vehicle-side data QD panel : Subsystem
      settings: PortSchema="{\"entries\":[{\"content\":{\"headerSize\":26,\"margin\":15,\"minimumSpacing\":25,\"sides\":[{\"content\":{\"connectorIds\":[\"In1\",\"In2\"]},\"type\":\"ConnectorPlacement.EquallySpacedRectSide\",\"uuid\":\"57d8a002-ec9a-4125-b797-7e7c6712bf02\"},{\"content\":{\"connectorIds\":[\"Out1\",\"Out2\"],\"side\":\"RIGHT\"},\"type\":\"ConnectorPlacement.EquallySpacedRectSide\",\"uuid\":\"9c166a96-12fc-4382-8ebe-da88da7fda26\"},{\"content\":{\"side\":\"TOP\"},\"type\":\"ConnectorPlacement.EquallySpacedRectSide\",\"uuid\":\"d709cb41-f5aa-4a2a-ad2b-35894222a9c1\"}]},\"type\":\"ConnectorPlacement.EquallySpacedConnector\",\"uuid\":\"04bb3772-118b-42d1-ac15-43c1b901053a\"}],\"packageUris\":[\"http://schema.mathworks.com/mf0/Connector/R2020b\"],\"version\":\"1.0\"}"
  Bus Element Out1 : Outport  PortName=IF-SDQ-GND-01
  Bus Element Out2 : Outport  Port=2  PortName=IF-SDQ-SCR-01
  wires:
  Vehicle-side data QD panel/2(IF-SDQ-SCR-01) -> Bus Element Out2/1
  Bus Element In2/1 -> Vehicle-side data QD panel/1(IF-STA-SDQ-01)
  Bus Element In1/1 -> Vehicle-side data QD panel/2(IF-GND-SDQ-01)
  Vehicle-side data QD panel/1(IF-SDQ-GND-01) -> Bus Element Out1/1

== system StarshipSystemModel/Starship/Communications/Ship/Relay link terminal ==
  Bus Element In1 : Inport  PortName=IF-GND-SRX-01
  Bus Element In2 : Inport  Port=2  PortName=IF-SLM-SRX-01
  Antenna aperture & radome : Subsystem
      settings: PortSchema="{\"entries\":[{\"content\":{\"headerSize\":26,\"margin\":15,\"minimumSpacing\":25,\"sides\":[{\"content\":{\"connectorIds\":[\"LConn1\"]},\"type\":\"ConnectorPlacement.EquallySpacedRectSide\",\"uuid\":\"57d8a002-ec9a-4125-b797-7e7c6712bf02\"},{\"content\":{\"connectorIds\":[\"RConn1\",\"Out1\"],\"side\":\"RIGHT\"},\"type\":\"ConnectorPlacement.EquallySpacedRectSide\",\"uuid\":\"9c166a96-12fc-4382-8ebe-da88da7fda26\"},{\"content\":{\"side\":\"TOP\"},\"type\":\"ConnectorPlacement.EquallySpacedRectSide\",\"uuid\":\"d709cb41-f5aa-4a2a-ad2b-35894222a9c1\"}]},\"type\":\"ConnectorPlacement.EquallySpacedConnector\",\"uuid\":\"04bb3772-118b-42d1-ac15-43c1b901053a\"}],\"packageUris\":[\"http://schema.mathworks.com/mf0/Connector/R2020b\"],\"version\":\"1.0\"}"
  RF/optical transceiver unit : Subsystem
      settings: PortSchema="{\"entries\":[{\"content\":{\"headerSize\":26,\"margin\":15,\"minimumSpacing\":25,\"sides\":[{\"content\":{\"connectorIds\":[\"In1\",\"LConn1\",\"In2\",\"LConn2\"]},\"type\":\"ConnectorPlacement.EquallySpacedRectSide\",\"uuid\":\"57d8a002-ec9a-4125-b797-7e7c6712bf02\"},{\"content\":{\"connectorIds\":[\"Out1\"],\"side\":\"RIGHT\"},\"type\":\"ConnectorPlacement.EquallySpacedRectSide\",\"uuid\":\"9c166a96-12fc-4382-8ebe-da88da7fda26\"},{\"content\":{\"side\":\"TOP\"},\"type\":\"ConnectorPlacement.EquallySpacedRectSide\",\"uuid\":\"d709cb41-f5aa-4a2a-ad2b-35894222a9c1\"}]},\"type\":\"ConnectorPlacement.EquallySpacedConnector\",\"uuid\":\"04bb3772-118b-42d1-ac15-43c1b901053a\"}],\"packageUris\":[\"http://schema.mathworks.com/mf0/Connector/R2020b\"],\"version\":\"1.0\"}"
  IF-PWR-SRA-01 : PMIOPort  Side=Left  ConnectionType=Bus: ElectricalPower
  IF-PWR-SRX-01 : PMIOPort  Port=2  Side=Left  ConnectionType=Bus: ElectricalPower
  Bus Element Out1 : Outport  PortName=IF-SRX-GND-01
  Bus Element Out2 : Outport  Port=2  PortName=IF-SRX-SLM-01
  wires:
  Antenna aperture & radome/1(IF-SRX-SLM-01) -> Bus Element Out2/1
  Bus Element In1/1 -> RF/optical transceiver unit/1(IF-GND-SRX-01)
  Bus Element In2/1 -> RF/optical transceiver unit/2(IF-SLM-SRX-01)
  RF/optical transceiver unit/1(IF-SRX-GND-01) -> Bus Element Out1/1
  connections:
  Antenna aperture & radome/RConn1 -- RF/optical transceiver unit/LConn1
  IF-PWR-SRA-01/RConn1 -- Antenna aperture & radome/LConn1
  IF-PWR-SRX-01/RConn1 -- RF/optical transceiver unit/LConn2

== system StarshipSystemModel/Starship/GNC/Control Command & Allocation/Actuator // Subsystem Command Routing ==
  Bus Element In1 : Inport  PortName=IF-CAA-CRS-01
  IF-PWR-GNC-01 : PMIOPort  Side=Left  ConnectionType=Bus: ElectricalPower
  Bus Element Out9 : Outport  PortName=IF-GNC-SPR-01
  Bus Element Out8 : Outport  Port=2  PortName=IF-GNC-BPR-01
  Bus Element Out7 : Outport  Port=3  PortName=IF-GNC-SFC-01
  Bus Element Out6 : Outport  Port=4  PortName=IF-GNC-BFC-01
  Bus Element Out5 : Outport  Port=5  PortName=IF-GNC-RCT-01
  Bus Element Out4 : Outport  Port=6  PortName=IF-GNC-TVC-01
  Bus Element Out3 : Outport  Port=7  PortName=IF-GNC-SEC-01
  Bus Element Out2 : Outport  Port=8  PortName=IF-GNC-BEC-01
  Bus Element Out1 : Outport  Port=9  PortName=IF-CRS-FHM-01
  Bus Element Out10 : Outport  Port=10  PortName=IF-GNC-ACT-01

== system StarshipSystemModel/Starship/GNC/Control Command & Allocation/Command Shaping & Limiting ==
  Bus Element In1 : Inport  PortName=IF-CLM-CAS-01
  Bus Element Out1 : Outport  PortName=IF-CAS-CAA-01

== system StarshipSystemModel/Starship/GNC/Control Command & Allocation/Control Allocation ==
  Bus Element In1 : Inport  PortName=IF-CAS-CAA-01
  Bus Element Out1 : Outport  PortName=IF-CAA-CRS-01

== system StarshipSystemModel/Starship/GNC/Flight Control/Attitude // Rate Control ==
  Bus Element In2 : Inport  PortName=IF-GPH-CAT-01
  Bus Element In1 : Inport  Port=2  PortName=IF-NSE-CAT-01
  Bus Element In3 : Inport  Port=3  PortName=IF-CAM-CAT-01
  Bus Element Out1 : Outport  PortName=IF-CAT-CLM-01

== system StarshipSystemModel/Starship/GNC/Flight Control/Control-Law Monitoring & Limiting ==
  Bus Element In2 : Inport  PortName=IF-CTR-CLM-01
  Bus Element In1 : Inport  Port=2  PortName=IF-CAT-CLM-01
  Bus Element Out1 : Outport  PortName=IF-CLM-CAS-01

== system StarshipSystemModel/Starship/GNC/Flight Control/Control-Mode Management ==
  Bus Element In1 : Inport  PortName=IF-FMG-CAM-01
  Bus Element Out1 : Outport  PortName=IF-CAM-CAT-01
  Bus Element Out2 : Outport  Port=2  PortName=IF-CAM-CTR-01

== system StarshipSystemModel/Starship/GNC/Flight Control/Trajectory // Translational Control ==
  Bus Element In1 : Inport  PortName=IF-NSE-CTR-01
  Bus Element In2 : Inport  Port=2  PortName=IF-GPH-CTR-01
  Bus Element In3 : Inport  Port=3  PortName=IF-CAM-CTR-01
  Bus Element Out1 : Outport  PortName=IF-CTR-CLM-01

== system StarshipSystemModel/Starship/GNC/GNC Flight Software & Mode Management/GNC Data & Interface Management ==
  Bus Element In2 : Inport  PortName=IF-BCR-GNC-01
  Bus Element In1 : Inport  Port=2  PortName=IF-SCR-GNC-01
  Bus Element In3 : Inport  Port=3  PortName=IF-TVC-GNC-01
  Bus Element Out1 : Outport  PortName=IF-FDB-FEX-01
  Bus Element Out2 : Outport  Port=2  PortName=IF-GNC-BTA-01
  Bus Element Out3 : Outport  Port=3  PortName=IF-GNC-STA-01

== system StarshipSystemModel/Starship/GNC/GNC Flight Software & Mode Management/GNC Function Execution ==
  Bus Element In1 : Inport  PortName=IF-FDB-FEX-01
  Bus Element Out1 : Outport  PortName=IF-FEX-FMG-01

== system StarshipSystemModel/Starship/GNC/GNC Flight Software & Mode Management/GNC Health Monitoring // Fault Response ==
  Bus Element In3 : Inport  PortName=IF-SAF-FHM-01
  Bus Element In1 : Inport  Port=2  PortName=IF-NVI-FHM-01
  Bus Element In2 : Inport  Port=3  PortName=IF-CRS-FHM-01
  Bus Element Out1 : Outport  PortName=IF-FHM-FMG-01
  Bus Element Out2 : Outport  Port=2  PortName=IF-GNC-TMS-01
  Bus Element Out3 : Outport  Port=3  PortName=IF-FHM-SAF-01

== system StarshipSystemModel/Starship/GNC/GNC Flight Software & Mode Management/GNC Mode Management ==
  Bus Element In1 : Inport  PortName=IF-FEX-FMG-01
  Bus Element In2 : Inport  Port=2  PortName=IF-FHM-FMG-01
  Bus Element Out1 : Outport  PortName=IF-FMG-GMD-01
  Bus Element Out2 : Outport  Port=2  PortName=IF-FMG-CAM-01

== system StarshipSystemModel/Starship/GNC/Guidance & Trajectory Management/Flight-Phase Guidance ==
  Bus Element In1 : Inport  PortName=IF-NSE-GPH-01
  Bus Element In2 : Inport  Port=2  PortName=IF-GTR-GPH-01
  Bus Element In3 : Inport  Port=3  PortName=IF-GCM-GPH-01
  Bus Element In4 : Inport  Port=4  PortName=IF-GMD-GPH-01
  Bus Element Out1 : Outport  PortName=IF-GPH-CAT-01
  Bus Element Out2 : Outport  Port=2  PortName=IF-GPH-CTR-01

== system StarshipSystemModel/Starship/GNC/Guidance & Trajectory Management/Guidance Constraints & Targeting ==
  Bus Element Out1 : Outport  PortName=IF-GCM-GPH-01

== system StarshipSystemModel/Starship/GNC/Guidance & Trajectory Management/Guidance Mode // Transition Logic ==
  Bus Element In1 : Inport  PortName=IF-FMG-GMD-01
  Bus Element Out1 : Outport  PortName=IF-GMD-GPH-01

== system StarshipSystemModel/Starship/GNC/Guidance & Trajectory Management/Trajectory // Reference Management ==
  Bus Element Out1 : Outport  PortName=IF-GTR-GPH-01

== system StarshipSystemModel/Starship/GNC/Navigation & State Estimation/Measurement Processing ==
  Bus Element In1 : Inport  PortName=IF-TMS-GNC-01
  Bus Element Out1 : Outport  PortName=IF-NMP-NSE-01

== system StarshipSystemModel/Starship/GNC/Navigation & State Estimation/Navigation Aiding Integration ==
  Bus Element Out1 : Outport  PortName=IF-NAI-NSE-01

== system StarshipSystemModel/Starship/GNC/Navigation & State Estimation/Navigation Validity & Integrity ==
  Bus Element In1 : Inport  PortName=IF-NSE-NVI-01
  Bus Element Out1 : Outport  PortName=IF-NVI-FHM-01

== system StarshipSystemModel/Starship/GNC/Navigation & State Estimation/State Estimation ==
  Bus Element In3 : Inport  PortName=IF-POS-GNC-01
  Bus Element In2 : Inport  Port=2  PortName=IF-NAI-NSE-01
  Bus Element In1 : Inport  Port=3  PortName=IF-NMP-NSE-01
  Bus Element Out4 : Outport  PortName=IF-NSE-GPH-01
  Bus Element Out3 : Outport  Port=2  PortName=IF-NSE-CTR-01
  Bus Element Out2 : Outport  Port=3  PortName=IF-NSE-CAT-01
  Bus Element Out1 : Outport  Port=4  PortName=IF-NSE-NVI-01

== system StarshipSystemModel/Starship/Power & Electrical Energy/Distributed Energy Storage/Battery Energy Storage ==
  IF-BES-INV-01 : PMIOPort  Side=Right  ConnectionType=Bus: ElectricalPower

== system StarshipSystemModel/Starship/Power & Electrical Energy/Distributed Energy Storage/Battery Isolation & Protection ==
  Bus Element In1 : Inport  PortName=IF-PMC-BIP-01
  Bus Element Out1 : Outport  PortName=IF-BIP-PIS-01

== system StarshipSystemModel/Starship/Power & Electrical Energy/Distributed Energy Storage/Battery State Monitoring ==
  Bus Element Out1 : Outport  PortName=IF-BSM-PSM-01

== system StarshipSystemModel/Starship/Power & Electrical Energy/High-Voltage Distribution & Protection/Branch // Load Protection Interface ==
  IF-PWR-GNC-01 : PMIOPort  Side=Right  ConnectionType=Bus: ElectricalPower
  IF-PWR-STR-01 : PMIOPort  Port=2  Side=Right  ConnectionType=Bus: ElectricalPower
  IF-PWR-TMS-01 : PMIOPort  Port=3  Side=Right  ConnectionType=Bus: ElectricalPower
  IF-PWR-STA-01 : PMIOPort  Port=4  Side=Right  ConnectionType=Bus: ElectricalPower
  IF-PWR-BTA-01 : PMIOPort  Port=5  Side=Right  ConnectionType=Bus: ElectricalPower
  IF-PWR-SDX-01 : PMIOPort  Port=6  Side=Right  ConnectionType=Bus: ElectricalPower
  IF-PWR-BDX-01 : PMIOPort  Port=7  Side=Right  ConnectionType=Bus: ElectricalPower
  IF-PWR-SRX-01 : PMIOPort  Port=8  Side=Right  ConnectionType=Bus: ElectricalPower
  IF-PWR-BRX-01 : PMIOPort  Port=9  Side=Right  ConnectionType=Bus: ElectricalPower
  IF-PWR-SRA-01 : PMIOPort  Port=10  Side=Right  ConnectionType=Bus: ElectricalPower
  IF-PWR-BRA-01 : PMIOPort  Port=11  Side=Right  ConnectionType=Bus: ElectricalPower
  IF-PWR-SPR-01 : PMIOPort  Port=12  Side=Right  ConnectionType=Bus: ElectricalPower
  IF-PWR-SFC-01 : PMIOPort  Port=13  Side=Right  ConnectionType=Bus: ElectricalPower
  IF-PWR-RCT-01 : PMIOPort  Port=14  Side=Right  ConnectionType=Bus: ElectricalPower
  IF-PWR-TVC-01 : PMIOPort  Port=15  Side=Right  ConnectionType=Bus: ElectricalPower
  IF-PWR-BEC-01 : PMIOPort  Port=16  Side=Right  ConnectionType=Bus: ElectricalPower
  IF-PWR-SEC-01 : PMIOPort  Port=17  Side=Right  ConnectionType=Bus: ElectricalPower
  IF-PWR-BFC-01 : PMIOPort  Port=18  Side=Right  ConnectionType=Bus: ElectricalPower
  IF-PWR-BPR-01 : PMIOPort  Port=19  Side=Right  ConnectionType=Bus: ElectricalPower
  Bus Element Out1 : Outport  PortName=IF-BPI-PIS-01

== system StarshipSystemModel/Starship/Power & Electrical Energy/High-Voltage Distribution & Protection/HV Distribution Network ==
  IF-PCR-HDN-01 : PMIOPort  Side=Left  ConnectionType=Bus: ElectricalPower
  Bus Element Out1 : Outport  PortName=IF-HDN-PSM-01

== system StarshipSystemModel/Starship/Power & Electrical Energy/High-Voltage Distribution & Protection/HV Switching & Isolation ==
  Bus Element In1 : Inport  PortName=IF-PMC-HSI-01
  Bus Element Out1 : Outport  PortName=IF-HSI-PIS-01

== system StarshipSystemModel/Starship/Power & Electrical Energy/Power Conversion & Conditioning/Conversion Monitoring ==
  Bus Element Out1 : Outport  PortName=IF-PCM-PSM-01
